simulink model "dc_motor"  (R2026a)
settings: Solver=FixedStepDiscrete  StopTime=5  FixedStep=1e-5
libraries: fl_lib x6, nesl_utility x5, ee_lib x2
settings Model: Creator=User  LastModifiedBy=User

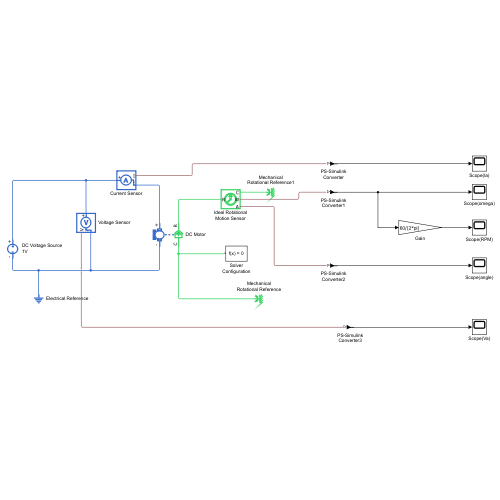
[thumbnail: Simulink's stored preview of the top-level diagram]
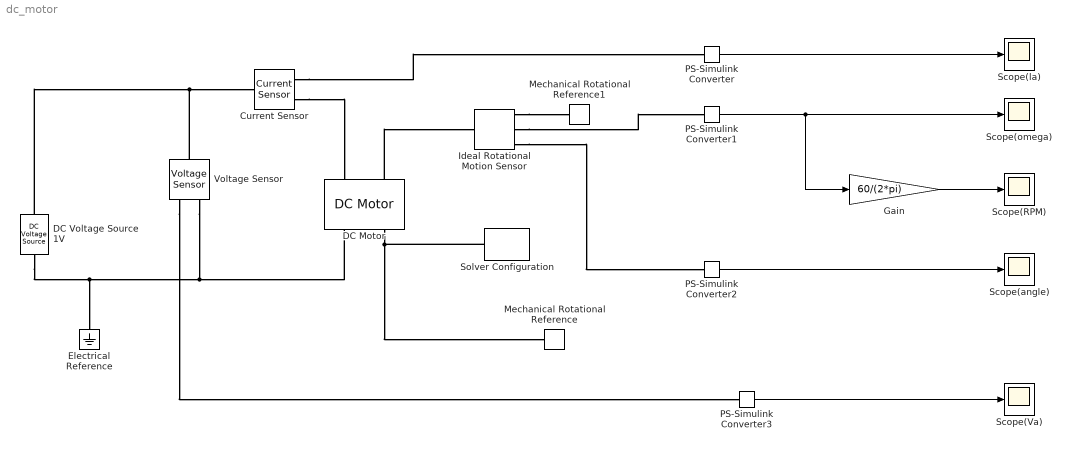
== system dc_motor ==
  Current Sensor : fl_lib/Electrical/Electrical Sensors/Current Sensor
  DC Motor : ee_lib/Electromechanical/Brushed Motors/DC Motor  field_option=ee.enum.field_option.pm  Rf=100 Ohm  Lf=1 H  Laf=0.15 H  If0=0 A  parameterization=ee.enum.dcparam_option.circuit_param  Ra=1 Ohm  La=1 H  emf_or_torque=ee.enum.emf_or_torque.kv  Kv=0.5 V*s/rad  Ki=6.876e-4 N*m/A  T_stall=0.24e-3 N*m  w_max=19100 rpm  w_rated=15000 rpm  P_rated=0.08 W  V_rated=1.5 V  lam_param=ee.enum.lam_param.damping  i_noload=0 A  V_i_noload=1.5 V  J=0.1 kg*m^2  lam=0.5 N*m*s/rad  speed0=0 rpm  alpha=3.93e-3 1/K  Tmeas=25 degC  thermal_mass=100 J/K  initial_temperature=25 degC
  DC Voltage Source 1V : ee_lib/Additional Components/SPICE Sources/DC Voltage Source  DC=1 V
  Electrical Reference : fl_lib/Electrical/Electrical Elements/Electrical Reference
  Gain : Gain  Gain=60/(2*pi)
  Ideal Rotational Motion Sensor : fl_lib/Mechanical/Mechanical Sensors/Ideal Rotational Motion Sensor  reference=foundation.enum.MeasurementReference.difference  acceleration_port=false  velocity_port=true  position_port=true  wrap_angle=false  offset=0 rad
  Mechanical Rotational Reference : fl_lib/Mechanical/Rotational Elements/Mechanical Rotational Reference
  Mechanical Rotational Reference1 : fl_lib/Mechanical/Rotational Elements/Mechanical Rotational Reference
  PS-Simulink Converter{,1..3} (4 alike) : nesl_utility/PS-Simulink Converter  PhysicalDomain=network_engine_domain  SubClassName=ps_output  LeftPortType=input  RightPortType=output  PseudoPeriodic=off  Frequencies=[]  VectorFormat=inherit  Unit=inherit  AffineConversion=off
  Scope(RPM) : Scope
      settings: DataLoggingVariableName=ScopeData2
  Scope(Va) : Scope
      settings: DataLoggingVariableName=ScopeData4
  Scope(angle) : Scope
      settings: DataLoggingVariableName=ScopeData3
  Scope(la) : Scope
      settings: ActiveDisplayYMinimum=-0.083320384722057758  ActiveDisplayYMaximum=0.74988347249851994
  Scope(omega) : Scope
      settings: ActiveDisplayYMinimum=-0.0833132581540294  ActiveDisplayYMaximum=0.74981932338626478
  Solver Configuration : nesl_utility/Solver Configuration  PhysicalDomain=network_engine_domain  SubClassName=solver  LeftPortType=input  RightPortType=generic  Tones=[]  Harmonics=[]  SimulateNoise=off  Profile=off  UseLocalSampling=off  EnableSwitchedLinearOptims=on  FrequencyDomain=off  UseCCode=off  RelTol=0.001  AbsTol=0.001  MinStep=1e-09  ToWorkspace=off  RevertToSquareIcSolve=off  NumHomotopyIterations=100  PhasorMode=off  PhasorModeNumHarmonics=1  ConsistencySolver=NEWTON_XTOL_AFTER_FTOL  CanonicalOrdering=CANONICAL  OptimizeIntermediates=OPTIMIZED  IndexReductionMethod=DerivativeReplacement  DoDC=off  ResidualTolerance=1e-09  ConsistencyTolSource=GLOBAL  ConsistencyAbsTol=0.001  ConsistencyRelTol=0.001  ConsistencyTolFactor=0.001  UseLocalSolver=on  LocalSolverChoice=NE_BACKWARD_EULER_ADVANCER  ResolveIndetEquations=on  FunctionEvalNumThread=1  LocalSolverSampleTime=1e-5  DoFixedCost=off  MaxNonlinIter=3  MaxModeIter=2  ComputeImpulses=off  ImpulseIterations=2  LinearAlgebra=auto  LinearAlgebraNumThread=0  EquationFormulation=NE_TIME_EF  DelaysMemoryBudget=1024  AutomaticFiltering=on  FilteringTimeConstant=0.001  PartitionStorageMethod=AS_NEEDED  PartitionMemoryBudget=1024  PartitionMethod=ROBUST  MultibodyUseLocalSolver=off  MultibodyLocalSolverChoice=ODE1  MultibodyLocalSolverSampleTime=0.001
  Voltage Sensor : fl_lib/Electrical/Electrical Sensors/Voltage Sensor
  wires:
  PS-Simulink Converter/1 -> Scope(la)/1
  PS-Simulink Converter1/1 -> Gain/1, Scope(omega)/1
  Gain/1 -> Scope(RPM)/1
  PS-Simulink Converter2/1 -> Scope(angle)/1
  PS-Simulink Converter3/1 -> Scope(Va)/1
  connections:
  DC Voltage Source 1V/RConn1 -- Electrical Reference/LConn1 -- Voltage Sensor/RConn2 -- DC Motor/RConn1
  DC Voltage Source 1V/LConn1 -- Voltage Sensor/LConn1 -- Current Sensor/LConn1
  Current Sensor/RConn2 -- DC Motor/LConn1
  DC Motor/LConn2 -- Ideal Rotational Motion Sensor/LConn1
  Ideal Rotational Motion Sensor/RConn1 -- Mechanical Rotational Reference1/LConn1
  DC Motor/RConn2 -- Solver Configuration/RConn1 -- Mechanical Rotational Reference/LConn1
  Current Sensor/RConn1 -- PS-Simulink Converter/LConn1
  Ideal Rotational Motion Sensor/RConn2 -- PS-Simulink Converter1/LConn1
  Ideal Rotational Motion Sensor/RConn3 -- PS-Simulink Converter2/LConn1
  Voltage Sensor/RConn1 -- PS-Simulink Converter3/LConn1
